simulink model "x1BLDCSpeedControl_EV_Layout_v2_fix"  (R2024b)
settings: Solver=ode23t  StartTime=0.0  StopTime=0.1  FixedStep=Ts  MaxStep=5e-4  RelTol=1e-3  EnableMultiTasking=on
PreLoadFcn:
  | BLDCSpeedControlData;
StartFcn:
  | % [EV_DAQ_V5_HOOK]
  | try; EV_DAQ_Builder_V5('AutoInit'); catch ME__daq; fprintf('[DAQ] Auto-init error: %s\n', ME__daq.message); end
StopFcn:
  | % [EV_DAQ_V5_HOOK]
  | try; EV_DAQ_Builder_V5('PostProcess'); catch ME__daq; fprintf('[DAQ] Post-process error: %s\n', ME__daq.message); end
values from neighbouring files (symbols this model uses):
  m = app.Rows(1:app.N, 1) >= 0.9*t    [EV_BlackBox_App.m]
  N = 0    [EV_BlackBox_App.m]
  p = inputParser    [Create_Simulation.m]    (also in EV_BlackBox_App.m = uipanel(parent, 'Title', title); Run_Simulation_Live.m; Run_Simulation_Log.m)
  s = regexprep(msg, '\s+', ' ')    [EV_BlackBox_App.m]    (also in Run_Simulation_Log.m = T.SOC(isfinite(T.SOC)))
undefined symbols (not defined in the file or in its folder): battery_builder_rtmsupport, cells_parallel, cells_series, DiscIntNeverNeededParam, Emax, Emax_thr, emf_max_ev, gcbh, I_cont, I_peak, Ke_ph, Kii, Kiv, Kiw, Kpi, Kpv, Kpw, load_scale, r_wheel, rpm_ramp, rpm_ref, T_Ifilt, Ts, Tsc, Vdc, Vlim_min, wheel_mass
libraries: nesl_utility x19, fl_lib x13, ee_lib x6, sm_lib x3, eeDiscretePi x2, Batteries2_lib x1, SignalEditorBlockLib x1, eePwmGenerator x1, eeGeneralControl x1
(part 2 of 2)

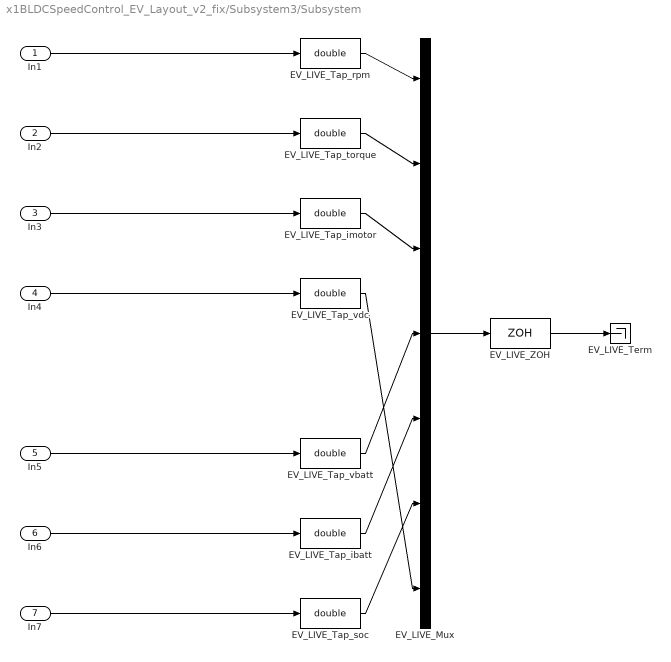
== system x1BLDCSpeedControl_EV_Layout_v2_fix/Subsystem3/Subsystem ==
  In1 : Inport
  In2 : Inport  Port=2
  In3 : Inport  Port=3
  In4 : Inport  Port=4
  In5 : Inport  Port=5
  In6 : Inport  Port=6
  In7 : Inport  Port=7
  EV_LIVE_Mux : Mux  Inputs=7
  EV_LIVE_Tap_ibatt : DataTypeConversion  OutDataTypeStr=double
  EV_LIVE_Tap_imotor : DataTypeConversion  OutDataTypeStr=double
  EV_LIVE_Tap_rpm : DataTypeConversion  OutDataTypeStr=double
  EV_LIVE_Tap_soc : DataTypeConversion  OutDataTypeStr=double
  EV_LIVE_Tap_torque : DataTypeConversion  OutDataTypeStr=double
  EV_LIVE_Tap_vbatt : DataTypeConversion  OutDataTypeStr=double
  EV_LIVE_Tap_vdc : DataTypeConversion  OutDataTypeStr=double
  EV_LIVE_Term : Terminator
  EV_LIVE_ZOH : ZeroOrderHold  SampleTime=0.1
  wires:
  EV_LIVE_ZOH/1 -> EV_LIVE_Term/1
  EV_LIVE_Tap_rpm/1 -> EV_LIVE_Mux/1
  EV_LIVE_Tap_vbatt/1 -> EV_LIVE_Mux/4
  EV_LIVE_Tap_soc/1 -> EV_LIVE_Mux/6
  EV_LIVE_Tap_ibatt/1 -> EV_LIVE_Mux/5
  EV_LIVE_Tap_vdc/1 -> EV_LIVE_Mux/7
  EV_LIVE_Tap_imotor/1 -> EV_LIVE_Mux/3
  EV_LIVE_Mux/1 -> EV_LIVE_ZOH/1
  In7/1 -> EV_LIVE_Tap_soc/1
  EV_LIVE_Tap_torque/1 -> EV_LIVE_Mux/2
  In5/1 -> EV_LIVE_Tap_vbatt/1
  In3/1 -> EV_LIVE_Tap_imotor/1
  In1/1 -> EV_LIVE_Tap_rpm/1
  In6/1 -> EV_LIVE_Tap_ibatt/1
  In4/1 -> EV_LIVE_Tap_vdc/1
  In2/1 -> EV_LIVE_Tap_torque/1

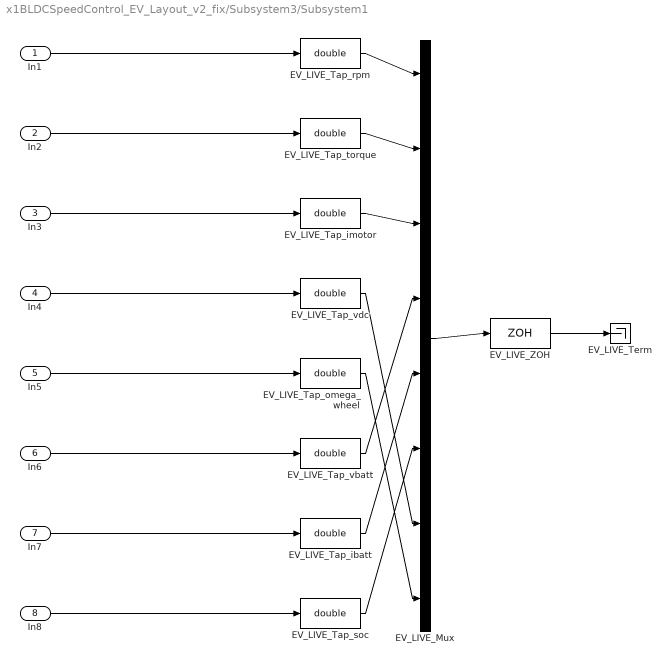
== system x1BLDCSpeedControl_EV_Layout_v2_fix/Subsystem3/Subsystem1 ==
  In1 : Inport
  In2 : Inport  Port=2
  In3 : Inport  Port=3
  In4 : Inport  Port=4
  In5 : Inport  Port=5
  In6 : Inport  Port=6
  In7 : Inport  Port=7
  In8 : Inport  Port=8
  EV_LIVE_Mux : Mux  Inputs=8
  EV_LIVE_Tap_ibatt : DataTypeConversion  OutDataTypeStr=double
  EV_LIVE_Tap_imotor : DataTypeConversion  OutDataTypeStr=double
  EV_LIVE_Tap_omega_wheel : DataTypeConversion  OutDataTypeStr=double
  EV_LIVE_Tap_rpm : DataTypeConversion  OutDataTypeStr=double
  EV_LIVE_Tap_soc : DataTypeConversion  OutDataTypeStr=double
  EV_LIVE_Tap_torque : DataTypeConversion  OutDataTypeStr=double
  EV_LIVE_Tap_vbatt : DataTypeConversion  OutDataTypeStr=double
  EV_LIVE_Tap_vdc : DataTypeConversion  OutDataTypeStr=double
  EV_LIVE_Term : Terminator
  EV_LIVE_ZOH : ZeroOrderHold  SampleTime=0.1
  wires:
  EV_LIVE_Tap_imotor/1 -> EV_LIVE_Mux/3
  EV_LIVE_ZOH/1 -> EV_LIVE_Term/1
  EV_LIVE_Tap_omega_wheel/1 -> EV_LIVE_Mux/8
  In3/1 -> EV_LIVE_Tap_imotor/1
  EV_LIVE_Tap_torque/1 -> EV_LIVE_Mux/2
  EV_LIVE_Tap_rpm/1 -> EV_LIVE_Mux/1
  EV_LIVE_Mux/1 -> EV_LIVE_ZOH/1
  EV_LIVE_Tap_soc/1 -> EV_LIVE_Mux/6
  In6/1 -> EV_LIVE_Tap_vbatt/1
  EV_LIVE_Tap_ibatt/1 -> EV_LIVE_Mux/5
  EV_LIVE_Tap_vdc/1 -> EV_LIVE_Mux/7
  EV_LIVE_Tap_vbatt/1 -> EV_LIVE_Mux/4
  In1/1 -> EV_LIVE_Tap_rpm/1
  In7/1 -> EV_LIVE_Tap_ibatt/1
  In5/1 -> EV_LIVE_Tap_omega_wheel/1
  In2/1 -> EV_LIVE_Tap_torque/1
  In4/1 -> EV_LIVE_Tap_vdc/1
  In8/1 -> EV_LIVE_Tap_soc/1

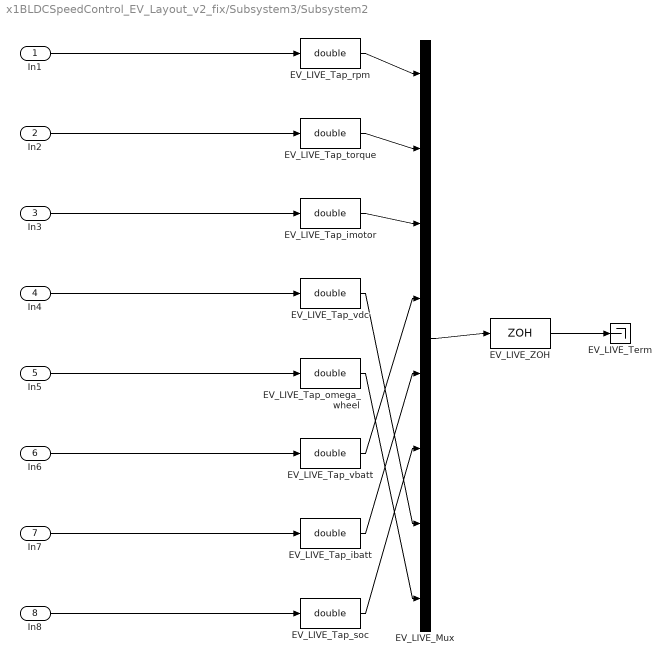
== system x1BLDCSpeedControl_EV_Layout_v2_fix/Subsystem3/Subsystem2 ==
  In1 : Inport
  In2 : Inport  Port=2
  In3 : Inport  Port=3
  In4 : Inport  Port=4
  In5 : Inport  Port=5
  In6 : Inport  Port=6
  In7 : Inport  Port=7
  In8 : Inport  Port=8
  EV_LIVE_Mux : Mux  Inputs=8
  EV_LIVE_Tap_ibatt : DataTypeConversion  OutDataTypeStr=double
  EV_LIVE_Tap_imotor : DataTypeConversion  OutDataTypeStr=double
  EV_LIVE_Tap_omega_wheel : DataTypeConversion  OutDataTypeStr=double
  EV_LIVE_Tap_rpm : DataTypeConversion  OutDataTypeStr=double
  EV_LIVE_Tap_soc : DataTypeConversion  OutDataTypeStr=double
  EV_LIVE_Tap_torque : DataTypeConversion  OutDataTypeStr=double
  EV_LIVE_Tap_vbatt : DataTypeConversion  OutDataTypeStr=double
  EV_LIVE_Tap_vdc : DataTypeConversion  OutDataTypeStr=double
  EV_LIVE_Term : Terminator
  EV_LIVE_ZOH : ZeroOrderHold  SampleTime=0.1
  wires:
  In4/1 -> EV_LIVE_Tap_vdc/1
  EV_LIVE_Mux/1 -> EV_LIVE_ZOH/1
  EV_LIVE_Tap_vdc/1 -> EV_LIVE_Mux/7
  EV_LIVE_Tap_vbatt/1 -> EV_LIVE_Mux/4
  EV_LIVE_Tap_rpm/1 -> EV_LIVE_Mux/1
  EV_LIVE_Tap_ibatt/1 -> EV_LIVE_Mux/5
  EV_LIVE_Tap_imotor/1 -> EV_LIVE_Mux/3
  EV_LIVE_ZOH/1 -> EV_LIVE_Term/1
  EV_LIVE_Tap_torque/1 -> EV_LIVE_Mux/2
  EV_LIVE_Tap_soc/1 -> EV_LIVE_Mux/6
  EV_LIVE_Tap_omega_wheel/1 -> EV_LIVE_Mux/8
  In1/1 -> EV_LIVE_Tap_rpm/1
  In5/1 -> EV_LIVE_Tap_omega_wheel/1
  In7/1 -> EV_LIVE_Tap_ibatt/1
  In8/1 -> EV_LIVE_Tap_soc/1
  In6/1 -> EV_LIVE_Tap_vbatt/1
  In3/1 -> EV_LIVE_Tap_imotor/1
  In2/1 -> EV_LIVE_Tap_torque/1

== system x1BLDCSpeedControl_EV_Layout_v2_fix/Sensing w a/Hall sensor/Subsystem ==
  theta : Inport
  Trigonometric Function : Trigonometry  Operator=sincos
  Trigonometric Function2 : Trigonometry  Operator=atan2
  mech->elec : Gain  Gain=p
  rad->deg : Gain  Gain=180/pi  SaturateOnIntegerOverflow=on  OutDataTypeStr=Inherit: Same as input  ParamDataTypeStr=Inherit: Same as input
  deg : Outport  VectorParamsAs1DForOutWhenUnconnected=off
  wires:
  Trigonometric Function2/1 -> rad->deg/1
  Trigonometric Function/1 -> Trigonometric Function2/1
  theta/1 -> mech->elec/1
  rad->deg/1 -> deg/1
  Trigonometric Function/2 -> Trigonometric Function2/2
  mech->elec/1 -> Trigonometric Function/1

== system x1BLDCSpeedControl_EV_Layout_v2_fix/Speed//RPM Controller/Commutation/Bit concatenate ==
  u : Inport
  Gain : Gain  Gain=[4 2 1]  Multiplication=Matrix(K*u)
  Sum of Elements : Sum  Inputs=+
  y : Outport  VectorParamsAs1DForOutWhenUnconnected=off
  wires:
  u/1 -> Gain/1
  Gain/1 -> Sum of Elements/1
  Sum of Elements/1 -> y/1
